simulink model "simple_manometer"  (R2025b)
settings: Solver=VariableStepAuto  StartTime=0.0  StopTime=3600  RelTol=1e-5  AbsTol=1e-7
libraries: nesl_utility x4, customization_lib x1
settings Model: PacingRate=5  Creator=degoede  LastModifiedBy=degoede
settings SolverCC: AutoScaleAbsTol=off
settings SimscapeCC: SimscapeNominalValues="[{\"value\":\"1\",\"unit\":\"A\"},{\"value\":\"10\",\"unit\":\"kPa\"},{\"value\":\"1\",\"unit\":\"cm^2\"},{\"value\":\"1\",\"unit\":\"cm^3/s\"},{\"value\":\"1\",\"unit\":\"kJ/kg\"},{\"value\":\"1\",\"unit\":\"kW\"},{\"value\":\"1\",\"unit\":\"l\"},{\"value\":\"1\",\"unit\":\"N\"},{\"value\":\"1\",\"unit\":\"N*m\"},{\"value\":\"1\",\"unit\":\"V\"},{\"value\":\"1e-4\",\"unit\":\"g/s\"}]"  SimscapeLogType=all  SimscapeLogSimulationStatistics=on  SimscapeLogOpenViewer=on  SimscapeLogLimitData=off

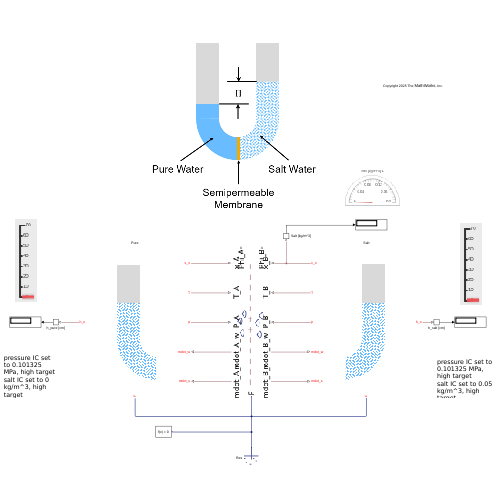
[thumbnail: Simulink's stored preview of the top-level diagram]
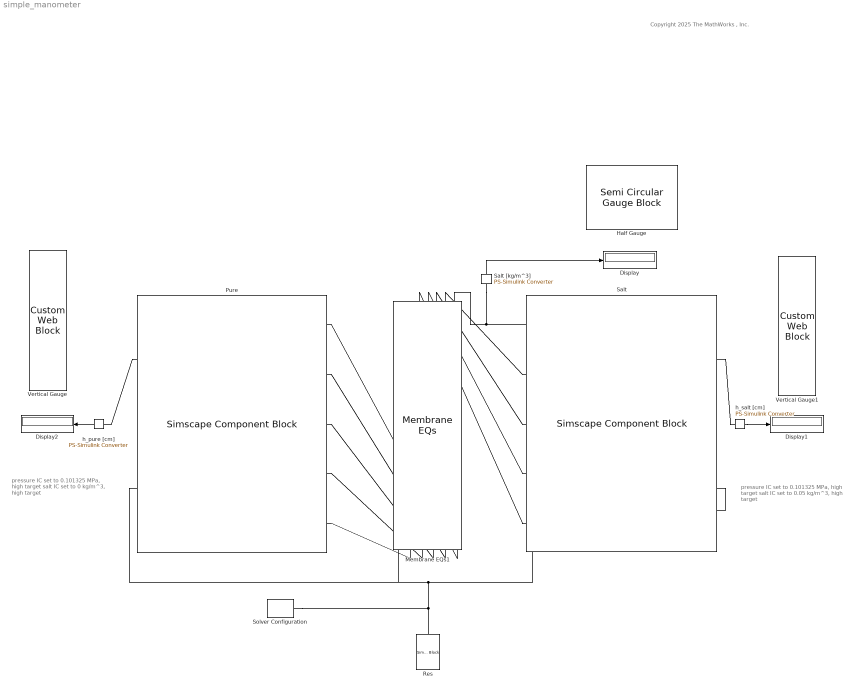
== system simple_manometer ==
  note: pressure IC set to 0.101325 MPa, high target
      | salt IC set to 0 kg/m^3, high target
  note: pressure IC set to 0.101325 MPa, high target
      | salt IC set to 0.05 kg/m^3, high target
  note: Copyright 2025 The MathWorks , Inc.
  Display : Display
  Display1 : Display
  Display2 : Display
  Half Gauge : SemiCircularGaugeBlock  ScaleMax=0.2  FontColor=[0.0, 0.0, 0.0]
  Membrane EQs1 : customization_lib/membranes/Membrane EQs  A_w=2.57e-6 m^3/(N*s)  B_s=2.30e-8 m/s  A_m=1 cm^2
      settings: SourceProductName=Customization  InternalSimscapePortConfiguration="{\"Bottom\":[{\"id\":\"mdot_B_x\",\"label\":\"mdot_B_x\",\"type\":\"output\"},{\"id\":\"mdot_B_w\",\"label\":\"mdot_B_w\",\"type\":\"output\"},{\"id\":\"P_B\",\"label\":\"P_B\",\"type\":\"input\"},{\"id\":\"T_B\",\"label\":\"T_B\",\"type\":\"input\"},{\"id\":\"x_B\",\"label\":\"x_B\",\"type\":\"input\"}],\"Left\":[{\"id\":\"F\",\"label\":\"F\",\"type\":\"customization.solution.solution\"}],\"Right\":[{\"id\":\"Phi_A\",\"label\":\"Phi_A\",\"type\":\"output\"},{\"id\":\"Phi_B\",\"label\":\"Phi_B\",\"type\":\"output\"}],\"Top\":[{\"id\":\"mdot_A_x\",\"label\":\"mdot_A_x\",\"type\":\"output\"},{\"id\":\"mdot_A_w\",\"label\":\"mdot_A_w\",\"type\":\"output\"},{\"id\":\"P_A\",\"label\":\"P_A\",\"type\":\"input\"},{\"id\":\"T_A\",\"label\":\"T_A\",\"type\":\"input\"},{\"id\":\"x_A\",\"label\":\"x_A\",\"type\":\"input\"}]}"
  Pure : SimscapeComponentBlock  SourceFile=simple_chamber  ComponentPath=simple_chamber  ComponentVariants="[\"simple_chamber\"]"  ComponentVariantNames="[\"simple_chamber\"]"  ClassName=simple_chamber  SchemaVersion=1  a_xsec=1 cm^2  x0=0 kg/m^3  p_atm=1.01325 bar  T0=293.15 K  h_specify=on  h_priority=High  h=0.5 m  h_nominal_specify=off  h_nominal_value=1  h_nominal_unit=m
      settings: CopyFcn=simscape.sscblock.internal.componentBlockCallback(gcbh,'COPY')  PreCopyFcn=simscape.sscblock.internal.componentBlockCallback(gcbh,'PRECOPY')  PreDeleteFcn=simscape.sscblock.internal.componentBlockCallback(gcbh,'PREDELETE')  InternalSimscapePortConfiguration="{\"Bottom\":[{\"id\":\"F\",\"label\":\"F\",\"type\":\"customization.solution.solution\"}],\"Left\":[{\"id\":\"x_o\",\"label\":\"x_o\",\"type\":\"output\"},{\"id\":\"T\",\"label\":\"T\",\"type\":\"output\"},{\"id\":\"p\",\"label\":\"p\",\"type\":\"output\"},{\"id\":\"mdot_w\",\"label\":\"mdot_w\",\"type\":\"input\"},{\"id\":\"mdot_s\",\"label\":\"mdot_s\",\"type\":\"input\"}],\"Right\":[{\"id\":\"h_o\",\"label\":\"h_o\",\"type\":\"output\"}],\"Top\":[]}"
      mask Type: Simple Chamber (SS)
  Res : SimscapeComponentBlock  SourceFile=customization.solution.elements.reservoir  ComponentPath=customization.solution.elements.reservoir  ComponentVariants="[\"customization.solution.elements.reservoir\"]"  ComponentVariantNames="[\"reservoir\"]"  ClassName=reservoir  SchemaVersion=1  pressure_spec=foundation.enum.pressure_spec.atmospheric  reservoir_pressure=0.101325 MPa  reservoir_temperature=293.15 K  reservoir_concentration=0 kg/m^3  area=pi cm^2
      settings: CopyFcn=simscape.sscblock.internal.componentBlockCallback(gcbh,'COPY')  PreCopyFcn=simscape.sscblock.internal.componentBlockCallback(gcbh,'PRECOPY')  PreDeleteFcn=simscape.sscblock.internal.componentBlockCallback(gcbh,'PREDELETE')  InternalSimscapePortConfiguration="{\"Bottom\":[],\"Left\":[{\"id\":\"A\",\"label\":\"A\",\"type\":\"customization.solution.solution\"}],\"Right\":[],\"Top\":[]}"
      mask Type: Reservoir (SS)
  Salt : SimscapeComponentBlock  SourceFile=simple_chamber  ComponentPath=simple_chamber  ComponentVariants="[\"simple_chamber\"]"  ComponentVariantNames="[\"simple_chamber\"]"  ClassName=simple_chamber  SchemaVersion=1  a_xsec=1 cm^2  x0=0.05 kg/m^3  p_atm=1.01325 bar  T0=293.15 K  h_specify=on  h_priority=High  h=0.5 m  h_nominal_specify=off  h_nominal_value=1  h_nominal_unit=m
      settings: CopyFcn=simscape.sscblock.internal.componentBlockCallback(gcbh,'COPY')  PreCopyFcn=simscape.sscblock.internal.componentBlockCallback(gcbh,'PRECOPY')  PreDeleteFcn=simscape.sscblock.internal.componentBlockCallback(gcbh,'PREDELETE')  InternalSimscapePortConfiguration="{\"Bottom\":[{\"id\":\"F\",\"label\":\"F\",\"type\":\"customization.solution.solution\"}],\"Left\":[{\"id\":\"x_o\",\"label\":\"x_o\",\"type\":\"output\"},{\"id\":\"T\",\"label\":\"T\",\"type\":\"output\"},{\"id\":\"p\",\"label\":\"p\",\"type\":\"output\"},{\"id\":\"mdot_w\",\"label\":\"mdot_w\",\"type\":\"input\"},{\"id\":\"mdot_s\",\"label\":\"mdot_s\",\"type\":\"input\"}],\"Right\":[{\"id\":\"h_o\",\"label\":\"h_o\",\"type\":\"output\"}],\"Top\":[]}"
      mask Type: Simple Chamber (SS)
  Salt [kg/m^3] : nesl_utility/PS-Simulink Converter  PhysicalDomain=network_engine_domain  SubClassName=ps_output  LeftPortType=input  RightPortType=output  PseudoPeriodic=off  Frequencies=[]  VectorFormat=inherit  Unit=kg/m^3  AffineConversion=off
  Solver Configuration : nesl_utility/Solver Configuration  PhysicalDomain=network_engine_domain  SubClassName=solver  LeftPortType=input  RightPortType=generic  Tones=[]  Harmonics=[]  SimulateNoise=off  Profile=off  UseLocalSampling=off  EnableSwitchedLinearOptims=on  FrequencyDomain=off  UseCCode=off  RelTol=0.001  AbsTol=0.001  MinStep=1e-09  ToWorkspace=off  RevertToSquareIcSolve=off  NumHomotopyIterations=100  PhasorMode=off  PhasorModeNumHarmonics=1  ConsistencySolver=NEWTON_XTOL_AFTER_FTOL  IndexReductionMethod=DerivativeReplacement  DoDC=off  ResidualTolerance=1e-09  ConsistencyTolSource=GLOBAL  ConsistencyAbsTol=0.001  ConsistencyRelTol=0.001  ConsistencyTolFactor=0.1  UseLocalSolver=off  LocalSolverChoice=NE_BACKWARD_EULER_ADVANCER  ResolveIndetEquations=on  FunctionEvalNumThread=1  LocalSolverSampleTime=0.001  DoFixedCost=off  MaxNonlinIter=3  MaxModeIter=2  ComputeImpulses=off  ImpulseIterations=2  LinearAlgebra=auto  LinearAlgebraNumThread=0  EquationFormulation=NE_TIME_EF  DelaysMemoryBudget=1024  AutomaticFiltering=off  FilteringTimeConstant=0.001  PartitionStorageMethod=AS_NEEDED  PartitionMemoryBudget=1024  PartitionMethod=ROBUST  MultibodyUseLocalSolver=off  MultibodyLocalSolverChoice=ODE1  MultibodyLocalSolverSampleTime=0.001
  Vertical Gauge : CustomWebBlock  LabelPosition=Hide  ShowInitialText=on  Configuration="{\"components\":[{\"name\":\"LinearScaleComponent\",\"settings\":{\"bounds\":{\"max\":70,\"min\":0,\"tickInterval\":\"auto\"},\"internalTickHeightScaleFactor\":0.5,\"labelColor\":[0,0,0],\"labelFont\":{\"font\":\"Arial\",\"fontSize\":12},\"labelOffset\":0.05,\"labelTransparency\":1,\"needleImage\":{\"size\":[21,75],\"src\":\"data:image\\/svg+xml;base64,PHN2ZyB4bWxucz0iaHR0cDovL3d3dy53My5vcmcvMjAwMC9zdmciIHhtbG5zOnhsaW5rPSJodHRwOi8vd3d3LnczLm9yZy8xOTk5L3hsaW5rIiB2aWV3Qm94PSIwIDAgMjEgNzUiPjxkZWZzPjxzdHlsZT4uY2xzLTF7ZmlsbDpub25lO30uY2xzLTJ7aXNvbGF0aW9uOmlzb2xhdGU7fS5jbHMtM3tjbGlwLXBhdGg6dXJsKCNjbGlwLXBhdGgpO30uY2xzLTR7b3BhY2l0eTowLjM7bWl4LWJsZW5kLW1vZGU6bXVsdGlwbHk7fS5jbHMtNXtmaWxsOiNlYjI2Mjk7fTwvc3R5bGU+PGNsaXBQYXRoIGlkPSJjbGlwLXBhdGgiIHRyYW5zZm9y ...(+1928 chars)\",\"srcOrientation\":\"horizontal\"},\"needleOffset\":[0.007413509060955519,0],\"needleSize\":{\"height\":0.11955094537815127,\"width\":0.7589285714285714},\"position\":[0.015821953781512604,0.06944444444444445,0.7996031746031746,0.9641544117647058],\"referencePoint\":\"auto\",\"scaleColors\":[],\"scaleColorsSize\":0.2,\"scaleDirection\":\"BT\",\"showLabels\":1,\"showMinorTicks\":0,\"showSpanLine\":1,\"showTicks\":1,\"tickColor\":[0,0,0],\"tickTransparency\":1,\"valueBarColor\":[38,140,221],\"valueBarOffset\":0,\"valueBarSize\":0.23,\"valueBarTransparency\":1}},{\"name\":\"BackgroundImageComponent\",\"settings\":{\"image\":{\"size\":[380,101],\"src\":\"data:image\\/svg+xml;base64,PHN2ZyBpZD0iZnJhbWUiIHhtbG5zPSJodHRwOi8vd3d3LnczLm9yZy8yMDAwL3N2ZyIgeG1sbnM6eGxpbms9Imh0dHA6Ly93d3cudzMub3JnLzE5OTkveGxpbmsiIHZpZXdCb3g9IjAgMCAzODAgMTAxIj48ZGVmcz48c3R5bGU+LmNscy0xe2ZpbGw6IzAwMmI0Mjt9LmNscy0ye2ZpbGw6IzQyNzA4Mjt9LmNscy0ze2ZpbGw6dXJsKCNyYWRpYWwtZ3JhZGllbnQpO308L3N0eWxlPjxyYWRpYWxHcmFkaWVudCBpZD0icmFkaWFsLWdyYWRpZW50IiBjeD0iMTkwIiBjeT0iNTAuNSIgcj0iMjY5LjIxIiBncmFkaWVudFVuaXRzPSJ1c2VyU3BhY2VPblVzZSI+PHN0b3Agb2Zmc2V0PSIwLjAxIiBzdG9wLWNvbG9yPSIjM2U0ZjU4Ii8+PHN0b3Agb2Zmc2V0PSIwLjA2IiBzdG9wLWNvbG9yPSIjNDQ1NzYxIi8+PHN0b3Agb2Zmc2V0PSIwLjE1IiBzdG9wLWNvbG9yPSIjNTU2YTc2Ii8+PHN0b3Agb2Zmc2V0PSIwLjI1IiBzdG9wLWNvbG9yPSIjNmQ4ODk1Ii8+PHN0b3Agb2Zmc2V0PSIwLjM4IiBzdG9wLWNvbG9yPSIjOGZiMmMzIi8+PHN0b3Agb2Zmc2V0PSIwLjUyIiBzdG9wLWNvbG9yPSIjYjZlNGZhIi8+PHN0b3Agb2Zmc2V0PSIxIiBzdG9wLWNvbG9yPSIjMTU0NjU3Ii8+PC9yYWRpYWxHcmFkaWVudD48L2RlZnM+PGcgaWQ9IkxheWVyXzIiIGRhdGEtbmFtZT0iTGF5ZXIgMiI+PGcgaWQ9IkxheWVyXzEtMiIgZGF0YS1uYW1lPSJMYXllciAxLTIiPjxyZWN0IGlkPSJyZWN0MTAzNiIgY2xhc3M9ImNscy0xIiB4PSIxMSIgeT0iMTEiIHdpZHRoPSIzNTgiIGhlaWdodD0iNzkiLz48cGF0aCBpZD0icGF0aDEwMzgiIGNsYXNzPSJjbHMtMiIgZD0iTTgsOFY5M0gzNzJWOFpNMzY5LDkwSDExVjExSDM2OVoiLz48cGF0aCBpZD0icGF0aDEwNDAiIGNsYXNzPSJjbHMtMyIgZD0iTTAsMFYxMDFIMzgwVjBaTTM3Miw5M0g4VjhIMzcyWiIvPjwvZz48L2c+PC9zdmc+\",\"srcOrientation\":\"horizontal\"},\"position\":[0,0,1,1],\"scaleMode\":\"0\"}},{\"name\":\"ForegroundImageComponent\",\"settings\":{\"image\":{\"size\":[0,0],\"src\":\"default\",\"srcOrientation\":[]},\"isForeground\":1,\"position\":[0,0,1,1],\"scaleMode\":\"0\"}}],\"derived\":{\"blockParameters\":{\"ForegroundColor\":[0,0,0],\"Limits\":{\"Max\":70,\"Min\":0,\"Ticks\":\"auto\"},\"ScaleColors\":[],\"ScaleDirection\":\"Clockwise\",\"ScaleMax\":70,\"ScaleMin\":0,\"TickInterval\":\"auto\",\"fixedAspectRatio\":\"on\"}},\"settings\":{\"BindingType\":\"signal\",\"backgroundColor\":[0,0,0,\"1\"],\"backgroundOffset\":0,\"backgroundOpacity\":1,\"fixedAspectRatio\":\"on\",\"orientation\":\"vertical\",\"showBackgroundColor\":false,\"value\":0,\"version\":\"R2023a\"},\"type\":\"LinearGauge\"}"  CustomBackgroundColor="{\"color\":[0.9019607843137255,0.9019607843137255,0.9019607843137255],\"show\":true}"
  Vertical Gauge1 : CustomWebBlock  LabelPosition=Hide  ShowInitialText=on  Configuration="{\"components\":[{\"name\":\"LinearScaleComponent\",\"settings\":{\"bounds\":{\"max\":70,\"min\":0,\"tickInterval\":\"auto\"},\"internalTickHeightScaleFactor\":0.5,\"labelColor\":[0,0,0],\"labelFont\":{\"font\":\"Arial\",\"fontSize\":12},\"labelOffset\":0.05,\"labelTransparency\":1,\"needleImage\":{\"size\":[21,75],\"src\":\"data:image\\/svg+xml;base64,PHN2ZyB4bWxucz0iaHR0cDovL3d3dy53My5vcmcvMjAwMC9zdmciIHhtbG5zOnhsaW5rPSJodHRwOi8vd3d3LnczLm9yZy8xOTk5L3hsaW5rIiB2aWV3Qm94PSIwIDAgMjEgNzUiPjxkZWZzPjxzdHlsZT4uY2xzLTF7ZmlsbDpub25lO30uY2xzLTJ7aXNvbGF0aW9uOmlzb2xhdGU7fS5jbHMtM3tjbGlwLXBhdGg6dXJsKCNjbGlwLXBhdGgpO30uY2xzLTR7b3BhY2l0eTowLjM7bWl4LWJsZW5kLW1vZGU6bXVsdGlwbHk7fS5jbHMtNXtmaWxsOiNlYjI2Mjk7fTwvc3R5bGU+PGNsaXBQYXRoIGlkPSJjbGlwLXBhdGgiIHRyYW5zZm9y ...(+1928 chars)\",\"srcOrientation\":\"horizontal\"},\"needleOffset\":[0.007413509060955519,0],\"needleSize\":{\"height\":0.11955094537815127,\"width\":0.7589285714285714},\"position\":[0.015821953781512604,0.06944444444444445,0.7996031746031746,0.9641544117647058],\"referencePoint\":\"auto\",\"scaleColors\":[],\"scaleColorsSize\":0.2,\"scaleDirection\":\"BT\",\"showLabels\":1,\"showMinorTicks\":0,\"showSpanLine\":1,\"showTicks\":1,\"tickColor\":[0,0,0],\"tickTransparency\":1,\"valueBarColor\":[108,244,255],\"valueBarOffset\":0,\"valueBarSize\":0.23,\"valueBarTransparency\":1}},{\"name\":\"BackgroundImageComponent\",\"settings\":{\"image\":{\"size\":[380,101],\"src\":\"data:image\\/svg+xml;base64,PHN2ZyBpZD0iZnJhbWUiIHhtbG5zPSJodHRwOi8vd3d3LnczLm9yZy8yMDAwL3N2ZyIgeG1sbnM6eGxpbms9Imh0dHA6Ly93d3cudzMub3JnLzE5OTkveGxpbmsiIHZpZXdCb3g9IjAgMCAzODAgMTAxIj48ZGVmcz48c3R5bGU+LmNscy0xe2ZpbGw6IzAwMmI0Mjt9LmNscy0ye2ZpbGw6IzQyNzA4Mjt9LmNscy0ze2ZpbGw6dXJsKCNyYWRpYWwtZ3JhZGllbnQpO308L3N0eWxlPjxyYWRpYWxHcmFkaWVudCBpZD0icmFkaWFsLWdyYWRpZW50IiBjeD0iMTkwIiBjeT0iNTAuNSIgcj0iMjY5LjIxIiBncmFkaWVudFVuaXRzPSJ1c2VyU3BhY2VPblVzZSI+PHN0b3Agb2Zmc2V0PSIwLjAxIiBzdG9wLWNvbG9yPSIjM2U0ZjU4Ii8+PHN0b3Agb2Zmc2V0PSIwLjA2IiBzdG9wLWNvbG9yPSIjNDQ1NzYxIi8+PHN0b3Agb2Zmc2V0PSIwLjE1IiBzdG9wLWNvbG9yPSIjNTU2YTc2Ii8+PHN0b3Agb2Zmc2V0PSIwLjI1IiBzdG9wLWNvbG9yPSIjNmQ4ODk1Ii8+PHN0b3Agb2Zmc2V0PSIwLjM4IiBzdG9wLWNvbG9yPSIjOGZiMmMzIi8+PHN0b3Agb2Zmc2V0PSIwLjUyIiBzdG9wLWNvbG9yPSIjYjZlNGZhIi8+PHN0b3Agb2Zmc2V0PSIxIiBzdG9wLWNvbG9yPSIjMTU0NjU3Ii8+PC9yYWRpYWxHcmFkaWVudD48L2RlZnM+PGcgaWQ9IkxheWVyXzIiIGRhdGEtbmFtZT0iTGF5ZXIgMiI+PGcgaWQ9IkxheWVyXzEtMiIgZGF0YS1uYW1lPSJMYXllciAxLTIiPjxyZWN0IGlkPSJyZWN0MTAzNiIgY2xhc3M9ImNscy0xIiB4PSIxMSIgeT0iMTEiIHdpZHRoPSIzNTgiIGhlaWdodD0iNzkiLz48cGF0aCBpZD0icGF0aDEwMzgiIGNsYXNzPSJjbHMtMiIgZD0iTTgsOFY5M0gzNzJWOFpNMzY5LDkwSDExVjExSDM2OVoiLz48cGF0aCBpZD0icGF0aDEwNDAiIGNsYXNzPSJjbHMtMyIgZD0iTTAsMFYxMDFIMzgwVjBaTTM3Miw5M0g4VjhIMzcyWiIvPjwvZz48L2c+PC9zdmc+\",\"srcOrientation\":\"horizontal\"},\"position\":[0,0,1,1],\"scaleMode\":\"0\"}},{\"name\":\"ForegroundImageComponent\",\"settings\":{\"image\":{\"size\":[0,0],\"src\":\"default\",\"srcOrientation\":[]},\"isForeground\":1,\"position\":[0,0,1,1],\"scaleMode\":\"0\"}}],\"derived\":{\"blockParameters\":{\"ForegroundColor\":[0,0,0],\"Limits\":{\"Max\":70,\"Min\":0,\"Ticks\":\"auto\"},\"ScaleColors\":[],\"ScaleDirection\":\"Clockwise\",\"ScaleMax\":70,\"ScaleMin\":0,\"TickInterval\":\"auto\",\"fixedAspectRatio\":\"on\"}},\"settings\":{\"BindingType\":\"signal\",\"backgroundColor\":[0,0,0,\"1\"],\"backgroundOffset\":0,\"backgroundOpacity\":1,\"fixedAspectRatio\":\"on\",\"orientation\":\"vertical\",\"showBackgroundColor\":false,\"value\":0,\"version\":\"R2023a\"},\"type\":\"LinearGauge\"}"  CustomBackgroundColor="{\"color\":[0.9019607843137255,0.9019607843137255,0.9019607843137255],\"show\":true}"
  h_pure [cm] : nesl_utility/PS-Simulink Converter  PhysicalDomain=network_engine_domain  SubClassName=ps_output  LeftPortType=input  RightPortType=output  PseudoPeriodic=off  Frequencies=[]  VectorFormat=inherit  Unit=cm  AffineConversion=off
  h_salt [cm] : nesl_utility/PS-Simulink Converter  PhysicalDomain=network_engine_domain  SubClassName=ps_output  LeftPortType=input  RightPortType=output  PseudoPeriodic=off  Frequencies=[]  VectorFormat=inherit  Unit=cm  AffineConversion=off
  wires:
  Salt [kg/m^3]/1 -> Display/1
  h_salt [cm]/1 -> Display1/1
  h_pure [cm]/1 -> Display2/1
  connections:
  Res/LConn1 -- Solver Configuration/RConn1 -- Membrane EQs1/LConn1 -- Pure/RConn2 -- Salt/RConn2
  Membrane EQs1/LConn3 -- Pure/LConn4
  Membrane EQs1/LConn2 -- Pure/LConn5
  Membrane EQs1/LConn6 -- Pure/LConn1
  Membrane EQs1/LConn4 -- Pure/LConn3
  Membrane EQs1/RConn4 -- Salt/LConn4
  Membrane EQs1/RConn3 -- Salt/LConn5
  Membrane EQs1/RConn5 -- Salt/LConn3
  Salt/LConn1 -- Membrane EQs1/RConn7 -- Salt [kg/m^3]/LConn1
  Membrane EQs1/RConn6 -- Salt/LConn2
  Membrane EQs1/LConn5 -- Pure/LConn2
  Salt/RConn1 -- h_salt [cm]/LConn1
  h_pure [cm]/LConn1 -- Pure/RConn1
